simulink model "FAST_11To14_MPC"  (R2019a)
settings: Solver=FixedStepAuto  StartTime=0.0  StopTime=10*DT  FixedStep=DT  RelTol=1e-3
values from neighbouring files (symbols this model uses):
  Cq = 0.0 0.0 0.0 0.0 0.0 0.0 0.0 0.0 0.0 0.0 0.0 0.0 0.0 0.0 0.0 0.0 0.0 0.0 0.0 0.0 0.0 0.0 0.0 0.0 0.0 0.0 0.0 0.0 0.0 0.0 0.0 0.0 0.0 0.0 0.0 0.0 0.0 0.0 0.0 0.0 0.0 0.0 0.0 0.0 0.0 0.0 0.0 0.0 0.0 0.0 0.0 0.0 0.0 0.0 0.0 0.0 0.0 0.0 0.0 0.0 0.0 0.0 0.0 0.0 0.0 0.0 0.0 0.0 0.0 0.0 0.0 0.0 0.0 0.0 0.0 0.0 0.0 0.0 0.0 0.0 0.0 0.0 0.0 0.0 0.0 0.0 0.0 0.0 0.0 0.0 0.0 0.0 0.0 0.0 0.0 0.0 0.0 0.0 0.0 0.0    [DD_test.sldd]    (also in testOutList.m = saveVarsMat.Cq)
  Drivetrain = struct    [dataDLR.m]
  DT = 0.008    [dataDLR.m]    (also in generateReport.m; initLPVParam.m; initWorkspace.m; runCalculateEvalCriteria.m)
  Lin_points : value not decoded    [DD_test.sldd]
  mu_old = zeros(2*N*nu,1)    [testCtrl.m]
  Ng = 97    [dataDLR.m]    (also in testCtrl.m)
  omegabar = interp1(Lin_points.V,Lin_points.RSpeed,Vbar,'spline')    [testCtrl.m]
  OutList = OutTable.Properties.VariableNames    [initLPVParam.m]    (also in testCtrl.m; testOutList.m = cell(40, 1); testqLPV.m = cell(40, 1))
  U = zeros(2*N,1)    [testCtrl.m]
  xk = Xk(nxa+1:2*nxa)    [testCtrl.m]
  Xko = kron(ones(N,1),xk)    [testCtrl.m]
undefined symbols (not defined in the file or in its folder): Rotor_Lambda, Rotor_Lamda, Rotor_Pitch, strmatch
libraries: MdlLib_ProcessOutput x1
settings Model: ExtModeTrigMode=oneshot  ExtModeArmWhenConnect=off  Creator=Hazim Namik  LastModifiedBy=ditt_aj
settings DataIOCC: LimitDataPoints=on  SaveFormat=Array  ReturnWorkspaceOutputs=off
settings OptimizationCC: BlockReduction=off  BooleanDataType=off  LifeSpan=inf
settings DebuggingCC: SaveWithParameterizedLinksMsg=none  UnderspecifiedInitializationDetection=Classic  MergeDetectMultiDrivingBlocksExec=none  SignalResolutionControl=TryResolveAllWithWarning  SFUnexpectedBacktrackingDiag=warning  SFNoUnconditionalDefaultTransitionDiag=warning  SFExecutionAtInitializationDiag=none  ArithmeticOperatorsInVariantConditions=warning
settings HardwareCC: ProdBitPerPointer=32  ProdBitPerSizeT=32  ProdBitPerPtrDiffT=32  ProdLargestAtomicFloat=None  ProdIntDivRoundTo=Undefined  ProdEndianess=Unspecified  ProdWordSize=32  ProdHWDeviceType=32-bit Generic  TargetUnknown=on
settings ModelReferenceCC: PropagateSignalLabelsOutOfModel=off
settings SFSimCC: SimUseLocalCustomCode=off
settings RTWCC: RTWUseLocalCustomCode=off
settings CodeAppCC: StateflowObjectComments=on
settings GRTTargetCC: TargetLangStandard=C89/C90 (ANSI)  GeneratePreprocessorConditionals=Disable all
settings ConfigComp: CovMetricSettings=dw  CovHtmlReporting=on  CovSaveCumulativeToWorkspaceVar=on  CovSaveSingleToWorkspaceVar=on  CovExternalEMLEnable=off

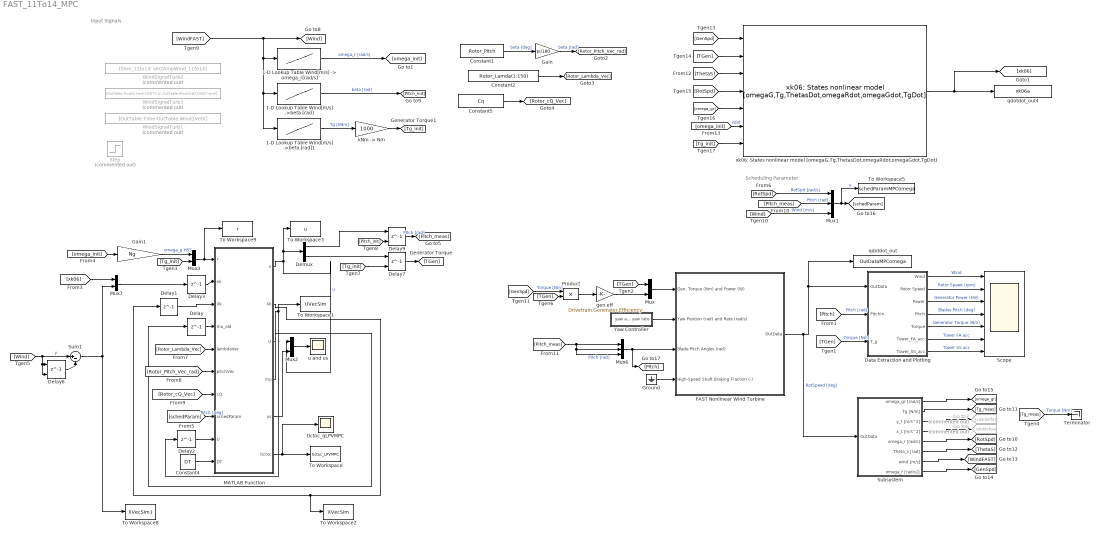
== system FAST_11To14_MPC ==
  note: Input Signals
  note: Scheduling Parameter
  "1-D Lookup Table Wind[m/s] -> omega_r[rad/s]" : Lookup_n-D  NumberOfTableDimensions=1  BreakpointsForDimension1=Lin_points.V  BreakpointsForDimension2=Rotor_Lambda  Table=Lin_points.RSpeed  InternalRulePriority=Speed  RndMeth=Simplest  InputSameDT=on
  1-D Lookup Table Wind[m/s] ->beta [rad] : Lookup_n-D  NumberOfTableDimensions=1  BreakpointsForDimension1=Lin_points.V  BreakpointsForDimension2=Rotor_Lambda  Table=Lin_points.Pitch  InternalRulePriority=Speed  RndMeth=Simplest  InputSameDT=on
  1-D Lookup Table Wind[m/s] ->beta [rad]1 : Lookup_n-D  NumberOfTableDimensions=1  BreakpointsForDimension1=Lin_points.V  BreakpointsForDimension2=Rotor_Lambda  Table=Lin_points.Torque  InternalRulePriority=Speed  RndMeth=Simplest  InputSameDT=on
  Constant1 : Constant  Value=Rotor_Pitch
  Constant2 : Constant  Value=Rotor_Lamda(1:150)
  Constant4 : Constant  Value=DT
  Constant5 : Constant  Value=Cq
  Data Extraction and Plotting : Subsystem
  Delay : Delay  DelayLength=1  InitialCondition=mu_old
  Delay1 : Delay  DelayLength=1  InitialCondition=Xko
  Delay2 : Delay  DelayLength=1  InitialCondition=U
  Delay3 : Delay  DelayLength=1  InitialCondition=xk
  Delay6 : Delay  DelayLength=1  InitialConditionSource=Input port  InitialCondition=[0, Lin_points.Torque(1)]
      settings: InputPortMap=u0,p4
  Delay7 : Delay  DelayLength=1  InitialConditionSource=Input port  InitialCondition=[0,omegabar]
      settings: InputPortMap=u0,p4
  Delay9 : Delay  DelayLength=1  InitialConditionSource=Input port  InitialCondition=[0,omegabar]
      settings: InputPortMap=u0,p4
  Demux : Demux  Outputs=2
  FAST Nonlinear Wind Turbine : Subsystem  mask(FAST Nonlinear Wind Turbine){}
      mask help: This block contains the FAST S-Function.
      mask init:
      | clear FAST_SFunc
  Gain : Gain  Gain=pi/180
  Gain1 : Gain  Gain=Ng
  Go to6 : Goto  Commented=on  GotoTag=xdotdotsw
  Go to7 : Goto  Commented=on  GotoTag=xdotdotfa
  Ground : Ground
  MATLAB Function : MATLAB Function  TreatAsAtomicUnit=on
  Mux{,2..3,7} (4 alike) : Mux  Inputs=2
  Mux1 : Mux  Inputs=3
  Mux6 : Mux  Inputs=3
  Product : Product  RndMeth=Zero
  Scope : Scope  NumInputPorts=7
      settings: Tag=Scope
  Step : Step  Commented=on  Time=0  Before=9.9960  After=11  SampleTime=0
  Subsystem : Subsystem
  Sum1 : Sum  Inputs=|+-
  Terminator : Terminator
  To Workspace : ToWorkspace  VariableName=tictoc_LPVMPC  SaveFormat=Timeseries  SampleTime=-1
  To Workspace1 : ToWorkspace  VariableName=UVecSim  SampleTime=-1
  To Workspace2 : ToWorkspace  VariableName=XVecSim  SampleTime=-1
  To Workspace3 : ToWorkspace  VariableName=u  SampleTime=-1
  To Workspace5 : ToWorkspace  VariableName=schedParamMPComega  SampleTime=-1
      settings: Save2DSignal=2-D array (concatenate along first dimension)
  To Workspace8 : ToWorkspace  VariableName=XVecSim1  SampleTime=-1
  To Workspace9 : ToWorkspace  VariableName=r  SampleTime=-1
  WindSignalTurb1 : FromWorkspace  Commented=on  VariableName=[OutTable.Time OutTable.Wind1VelX]  SampleTime=DT  OutputAfterFinalValue=Holding final value
  WindSignalTurb2 : FromWorkspace  Commented=on  VariableName=[time_11to14' vectAmpWind_11to14]  SampleTime=DT  OutputAfterFinalValue=Holding final value
  WindSignalTurb3 : FromWorkspace  Commented=on  VariableName=[OutTable.Time(1:(end-20/DT+1)),OutTable.Wind1VelX(20/DT:end)]  SampleTime=DT  OutputAfterFinalValue=Holding final value
  Yaw Controller : Subsystem
  gen eff : Gain  Gain=Drivetrain.Generator.Efficiency
  "kNm -> Nm" : Gain  Gain=1000
  qdotdot_out : ToWorkspace  VariableName=OutDataMPComega  SampleTime=-1
  qdotdot_out4 : ToWorkspace  VariableName=xk06a  SampleTime=-1
  tictoc_qLPVMPC : Scope
  u and us : Scope
  xk06: States nonlinear model [omegaG,Tg,ThetasDot,omegaRdot,omegaGdot,TgDot] : MdlLib_ProcessOutput/xk06: States nonlinear model [omegaG,Tg,ThetasDot,omegaRdot,omegaGdot,TgDot]  SystemSampleTime=-1
  wires:
  Mux/1 -> FAST Nonlinear Wind Turbine/1(Gen. Torque (Nm) and Power (W))
  Yaw Controller/1(yaw and yaw rate) -> FAST Nonlinear Wind Turbine/2(Yaw Position (rad) and Rate (rad/s))
  gen eff/1 -> Mux/2
  Product/1 -> gen eff/1
  Data Extraction and Plotting/3(Power) -> Scope/3  "Generator Power (kW)"
  [Pitch] -> Data Extraction and Plotting/2(PitchIn)  "Pitch [rad]"
  Data Extraction and Plotting/1(Wind) -> Scope/1  "Wind"
  Data Extraction and Plotting/2(Rotor Speed) -> Scope/2  "Rotor Speed (rpm)"
  [TGen] -> Data Extraction and Plotting/3(T_g)  "Torque [Nm]"
  Data Extraction and Plotting/4(Pitch) -> Scope/4  "Blades Pitch (deg)"
  Data Extraction and Plotting/5(Torque) -> Scope/5  "Generator Torque (Nm)"
  Data Extraction and Plotting/6(Tower_FA_acc) -> Scope/6  "Tower FA acc"
  Data Extraction and Plotting/7(Tower_SS_acc) -> Scope/7  "Tower SS acc"
  Ground/1 -> FAST Nonlinear Wind Turbine/4(High-Speed Shaft Braking Fraction (-))
  [TGen] -> Mux/1
  Delay3/1 -> MATLAB Function/2(xk)
  Mux7/1 -> Delay3/1
  MATLAB Function/3(U) -> Delay2/1, To Workspace1/1
  [omega_init] -> Gain1/1
  Sum1/1 -> To Workspace8/1, Mux7/2
  Gain1/1 -> Mux3/1  "omega_g HSS"
  Mux3/1 -> To Workspace9/1, MATLAB Function/1(r)
  [Wind] -> Delay6/2, Delay6/1, Sum1/1  "y"
  Delay6/1 -> Sum1/2
  [xk06] -> Mux7/1
  [Rotor_cQ_Vec] -> MATLAB Function/7(cQ)
  MATLAB Function/1(u) -> Demux/1, To Workspace3/1, Mux2/1  "u"
  Delay1/1 -> MATLAB Function/3("Xk ")
  [Tg_init] -> Mux3/2
  MATLAB Function/2(Xk) -> Delay1/1, To Workspace2/1
  [schedParam] -> MATLAB Function/8(schedParam)  "Pitch [deg]"
  Delay2/1 -> MATLAB Function/9("U ")
  Constant4/1 -> MATLAB Function/10(DT)
  MATLAB Function/6(tictoc) -> tictoc_qLPVMPC/1, To Workspace/1
  [Rotor_Lambda_Vec] -> MATLAB Function/5(lambdaVec)
  [Rotor_Pitch_Vec_rad] -> MATLAB Function/6(pitchVec)
  MATLAB Function/4(mu) -> Delay/1
  Delay/1 -> MATLAB Function/4(mu_old)
  MATLAB Function/5(us) -> Mux2/2
  Mux2/1 -> u and us/1
  Constant5/1 -> [Rotor_cQ_Vec]
  Gain/1 -> [Rotor_Pitch_Vec_rad]  "beta [rad]"
  "1-D Lookup Table Wind[m/s] -> omega_r[rad/s]"/1 -> [omega_init]  "omega_r [rad/s]"
  Constant1/1 -> Gain/1  "beta [deg]"
  1-D Lookup Table Wind[m/s] ->beta [rad]/1 -> [Pitch_init]  "beta [rad]"
  [WindFAST] -> [Wind], "1-D Lookup Table Wind[m/s] -> omega_r[rad/s]"/1, 1-D Lookup Table Wind[m/s] ->beta [rad]/1, 1-D Lookup Table Wind[m/s] ->beta [rad]1/1
  1-D Lookup Table Wind[m/s] ->beta [rad]1/1 -> "kNm -> Nm"/1  "Tg [kNm]"
  "kNm -> Nm"/1 -> [Tg_init]
  Constant2/1 -> [Rotor_Lambda_Vec]
  FAST Nonlinear Wind Turbine/1(OutData) -> Subsystem/1(OutData), qdotdot_out/1, Data Extraction and Plotting/1(OutData)  "RotSpeed [deg]"
  Delay7/1 -> [TGen]
  [Tg_init] -> Delay7/2
  [Pitch_meas] -> Mux6/1, Mux6/3, Mux6/2  "Pitch [rad]"
  Mux6/1 -> [Pitch], FAST Nonlinear Wind Turbine/3(Blade Pitch Angles (rad))
  [Pitch_init] -> Delay9/2
  Demux/2 -> Delay7/1
  Demux/1 -> Delay9/1
  [TGen] -> Product/2
  [GenSpd] -> Product/1  "Torque [Nm]"
  Delay9/1 -> [Pitch_meas]  "Pitch [rad]"
  [GenSpd] -> xk06: States nonlinear model [omegaG,Tg,ThetasDot,omegaRdot,omegaGdot,TgDot]/1
  [TGen] -> xk06: States nonlinear model [omegaG,Tg,ThetasDot,omegaRdot,omegaGdot,TgDot]/2
  [ThetaS] -> xk06: States nonlinear model [omegaG,Tg,ThetasDot,omegaRdot,omegaGdot,TgDot]/3
  [RotSpd] -> xk06: States nonlinear model [omegaG,Tg,ThetasDot,omegaRdot,omegaGdot,TgDot]/4
  [omega_gr] -> xk06: States nonlinear model [omegaG,Tg,ThetasDot,omegaRdot,omegaGdot,TgDot]/5
  [omega_init] -> xk06: States nonlinear model [omegaG,Tg,ThetasDot,omegaRdot,omegaGdot,TgDot]/6  "xdot"
  [Tg_init] -> xk06: States nonlinear model [omegaG,Tg,ThetasDot,omegaRdot,omegaGdot,TgDot]/7
  xk06: States nonlinear model [omegaG,Tg,ThetasDot,omegaRdot,omegaGdot,TgDot]/1 -> [xk06], qdotdot_out4/1
  Subsystem/2(Tg [N/m]) -> [Tg_meas]
  Subsystem/8(omega_r [rad/s]1) -> [GenSpd]
  Subsystem/7(wind [m/s]) -> [WindFAST]
  Subsystem/6(Theta_s [rad]) -> [ThetaS]
  Subsystem/1(omega_gr [rad/s]) -> [omega_gr]
  Subsystem/3(y_t [m/s^2]) -> Go to7/1
  Subsystem/5(omega_r [rad/s]) -> [RotSpd]
  Subsystem/4(x_t [m/s^2]) -> Go to6/1
  [Tg_meas] -> Terminator/1  "Torque [Nm]"
  [Pitch_meas] -> Mux1/2  "Pitch [rad]"
  Mux1/1 -> To Workspace5/1, [schedParam]  "y"
  [RotSpd] -> Mux1/1  "RotSpd [rad/s]"
  [Wind] -> Mux1/3  "Wind [m/s]"

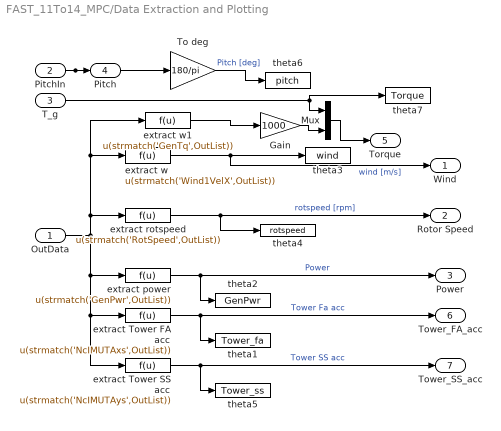
== system FAST_11To14_MPC/Data Extraction and Plotting ==
  OutData : Inport
  PitchIn : Inport  Port=2
  T_g : Inport  Port=3
  Gain : Gain  Gain=1000
  Mux : Mux  Inputs=2
  To deg : Gain  Gain=180/pi
  extract Tower FA acc : Fcn  Expr=u(strmatch('NcIMUTAxs',OutList))
  extract Tower SS acc : Fcn  Expr=u(strmatch('NcIMUTAys',OutList))
  extract power : Fcn  Expr=u(strmatch('GenPwr',OutList))
  extract rotspeed : Fcn  Expr=u(strmatch('RotSpeed',OutList))
  extract w : Fcn  Expr=u(strmatch('Wind1VelX',OutList))
  extract w1 : Fcn  Expr=u(strmatch('GenTq',OutList))
  theta1 : ToWorkspace  VariableName=Tower_fa  SampleTime=-1
      settings: MaxDataPoints=Inf  Decimation=3
  theta2 : ToWorkspace  VariableName=GenPwr  SampleTime=-1
      settings: MaxDataPoints=Inf  Decimation=3
  theta3 : ToWorkspace  VariableName=wind  SampleTime=-1
      settings: MaxDataPoints=Inf  Decimation=3
  theta4 : ToWorkspace  VariableName=rotspeed  SampleTime=-1
      settings: MaxDataPoints=Inf  Decimation=3
  theta5 : ToWorkspace  VariableName=Tower_ss  SampleTime=-1
      settings: MaxDataPoints=Inf  Decimation=3
  theta6 : ToWorkspace  VariableName=pitch  SampleTime=-1
      settings: MaxDataPoints=Inf  Decimation=3
  theta7 : ToWorkspace  VariableName=Torque  SampleTime=-1
      settings: MaxDataPoints=Inf  Decimation=3
  Wind : Outport
  Rotor Speed : Outport  Port=2
  Power : Outport  Port=3
  Pitch : Outport  Port=4
  Torque : Outport  Port=5
  Tower_FA_acc : Outport  Port=6
  Tower_SS_acc : Outport  Port=7
  wires:
  extract w/1 -> Wind/1, theta3/1  "wind [m/s]"
  extract rotspeed/1 -> theta4/1, Rotor Speed/1  "rotspeed [rpm]"
  extract power/1 -> theta2/1, Power/1  "Power"
  PitchIn/1 -> To deg/1, Pitch/1
  T_g/1 -> Mux/1, theta7/1
  extract Tower FA acc/1 -> theta1/1, Tower_FA_acc/1  "Tower Fa acc"
  OutData/1 -> extract w/1, extract w1/1, extract rotspeed/1, extract Tower SS acc/1, extract Tower FA acc/1, extract power/1
  extract Tower SS acc/1 -> theta5/1, Tower_SS_acc/1  "Tower SS acc"
  extract w1/1 -> Gain/1
  Gain/1 -> Mux/2
  Mux/1 -> Torque/1
  To deg/1 -> theta6/1  "Pitch [deg]"

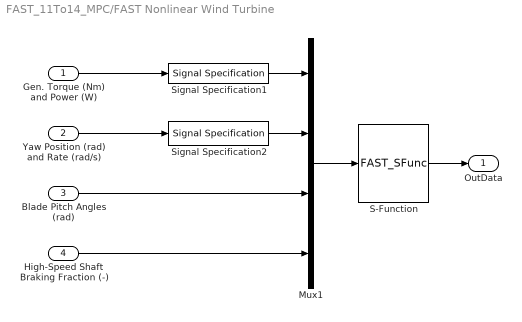
== system FAST_11To14_MPC/FAST Nonlinear Wind Turbine ==
  Gen. Torque (Nm) and Power (W) : Inport
  Yaw Position (rad) and Rate (rad/s) : Inport  Port=2
  Blade Pitch Angles (rad) : Inport  Port=3
  High-Speed Shaft Braking Fraction (-) : Inport  Port=4
  Mux1 : Mux
  S-Function : S-Function  FunctionName=FAST_SFunc  Parameters=FAST_InputFileName, TMax, 0  SFunctionDeploymentMode=off  EnableBusSupport=off
  Signal Specification1 : SignalSpecification  OutDataTypeStr=double  Dimensions=2
  Signal Specification2 : SignalSpecification  OutDataTypeStr=double  Dimensions=2
  OutData : Outport
  wires:
  Gen. Torque (Nm) and Power (W)/1 -> Signal Specification1/1
  S-Function/1 -> OutData/1
  Mux1/1 -> S-Function/1
  Blade Pitch Angles (rad)/1 -> Mux1/3
  Yaw Position (rad) and Rate (rad/s)/1 -> Signal Specification2/1
  Signal Specification1/1 -> Mux1/1
  Signal Specification2/1 -> Mux1/2
  High-Speed Shaft Braking Fraction (-)/1 -> Mux1/4

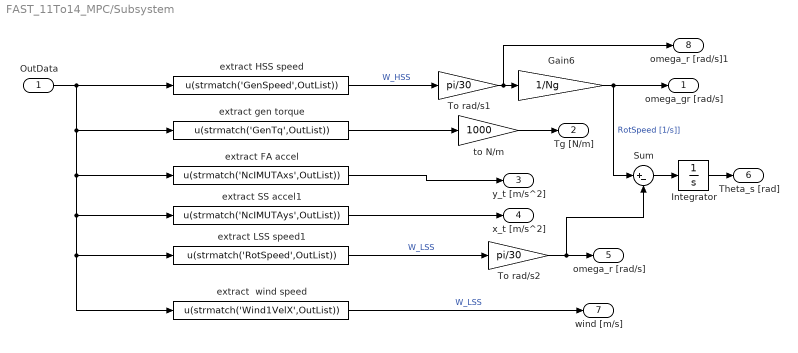
== system FAST_11To14_MPC/Subsystem ==
  OutData : Inport
  Gain6 : Gain  Gain=1/Ng
  Integrator : Integrator
  Sum : Sum  Inputs=|+-
  To rad/s1 : Gain  Gain=pi/30
  To rad/s2 : Gain  Gain=pi/30
  extract  wind speed : Fcn  Expr=u(strmatch('Wind1VelX',OutList))
  extract FA accel : Fcn  Expr=u(strmatch('NcIMUTAxs',OutList))
  extract HSS speed : Fcn  Expr=u(strmatch('GenSpeed',OutList))
  extract LSS speed1 : Fcn  Expr=u(strmatch('RotSpeed',OutList))
  extract SS accel1 : Fcn  Expr=u(strmatch('NcIMUTAys',OutList))
  extract gen torque : Fcn  Expr=u(strmatch('GenTq',OutList))
  to N/m : Gain  Gain=1000
  omega_gr [rad/s] : Outport
  Tg [N/m] : Outport  Port=2
  y_t [m/s^2] : Outport  Port=3
  x_t [m/s^2] : Outport  Port=4
  omega_r [rad/s] : Outport  Port=5
  Theta_s [rad] : Outport  Port=6
  wind [m/s] : Outport  Port=7
  omega_r [rad/s]1 : Outport  Port=8
  wires:
  to N/m/1 -> Tg [N/m]/1
  OutData/1 -> extract HSS speed/1, extract gen torque/1, extract  wind speed/1, extract LSS speed1/1, extract SS accel1/1, extract FA accel/1
  extract FA accel/1 -> y_t [m/s^2]/1
  extract HSS speed/1 -> To rad/s1/1  "W_HSS"
  extract gen torque/1 -> to N/m/1
  extract SS accel1/1 -> x_t [m/s^2]/1
  To rad/s1/1 -> omega_r [rad/s]1/1, Gain6/1
  extract LSS speed1/1 -> To rad/s2/1  "W_LSS"
  Gain6/1 -> omega_gr [rad/s]/1, Sum/1  "RotSpeed [1/s]]"
  To rad/s2/1 -> Sum/2, omega_r [rad/s]/1
  Sum/1 -> Integrator/1
  Integrator/1 -> Theta_s [rad]/1
  extract  wind speed/1 -> wind [m/s]/1  "W_LSS"

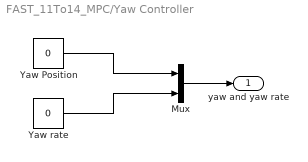
== system FAST_11To14_MPC/Yaw Controller ==
  Mux : Mux  Inputs=2
  Yaw Position : Constant  Value=0
  Yaw rate : Constant  Value=0
  yaw and yaw rate : Outport
  wires:
  Mux/1 -> yaw and yaw rate/1
  Yaw Position/1 -> Mux/1
  Yaw rate/1 -> Mux/2

== matlab function FAST_11To14_MPC/MATLAB Function ==
  settings: updateMethod=DISCRETE
  data: r input; u output; xk input; Xk input; mu_old input; lambdaVec input; pitchVec input; cQ input; schedParam input; U input; DT input; Xk output; U output; mu output; us output; tictoc output
function [u,Xk,U,mu,us,tictoc] = qLPVMPC_WECS(r,xk,Xk,mu_old,lambdaVec,pitchVec,cQ,schedParam,U,DT)
% MATLAB_Function calculates controller output u. It turns the QP into a 
% linear complementarity problem (LCP) and solves it with Lemke's algorithm.
%
% Inputs: * r: reference
%         * xk: quasiLPV KF state estimates
%         * Xk: Xko(= L*xk+S*U) delayed by one sample timestep
%         * mu_old: mu delayed by one sample timestep
%         * lambdaVec: lambda vector for cQ LUT 
%         * pitchVec: pitch vector for cQ LUT 
%         * cQ: torque coefficients LUT matrix
%         * schedParam: current values [omegaR, beta, V]
%         * U: U (from Xko = L*xk+S*U) delayed by one sample timestep
%
% Outputs: * u: controller output at current time step
%          * Xko: Future state trajectory (L*xk+S*U)
%          * U: Future input trajectory 
%          * mu: Result Lemke's algorithm/LCP: M mu +q >=0, mu>=0, mu'(Mmu+q)=0
%          * us: xuss(end) from xuss = [eye(4)-Ass -Bss;[1 0 0 0] 0]\[Bss*d;1]
%          * tictoc: tic-toc result

% Pablo S.G. Cisneros, Herbert Werner, ICS TUHH

%#codegen
coder.extrinsic('tic');
coder.extrinsic('toc');
tictoc = 0;
tic

%% Init N, Q, R
N = 40;
q_ = [1000 1 0 0*10^3 0*10^3 0 0]; %[10^4 0.1 1 1 100 0.1 0]; %q_ = [100 1000 1 0.01 0]; 7.351e+02 1.000e+00 1.938e+09 1.625e+08 1.491e+08 1.657e+03
r_ = [10^8 1]; %[10^7,0.1];
R_ = kron(eye(N),diag(r_)); %R_ = 1000*eye(N); 
p = 10*q_; %P = 1000*diag(q_);

Ulim = repmat([8 * pi/180, 20000]',2*N,1); %rate constraints 

Control_Pitch_Max = 90 /180 * pi;
Control_Pitch_Min = 0 /180 * pi;
Control_Torque_Limit = 47403;
Control_Torque_Min = 200;
schedParam(2) = min(max(schedParam(2), Control_Pitch_Min),Control_Pitch_Max);

% isBetaState = 0;
% nx = 4 + isBetaState; % number states plant: ThetaS,omegaR,omegaG,Tg
% ny = 2 + isBetaState; % number of outputs plant omegaG,Tg
nxA = 7;% nx + ny + 1; %number states augmented plant 
nu = 2; % plant inputs: Tg_ref, beta_ref

%% Shift Xk
Xk(1:end-nxA) = Xk(nxA+1:end); 
%Xk(1:nxA)

%% Calculate input u_dot_s = 0  and steady state x = r
us = [0;0]; %xuss(nxA+1:nxA+2); % xuss = [eye(size(Ass))-Ass -Bss;[1 0 0 0] 0] \ [Bss*d;reference];

iterations = 1; % omega_ref(Vest), Tg_ref(Vest)
refVec = zeros(nxA,1);
refVec(1:2) = r;
ref = repmat(refVec,N,1); %ref = kron(ones(N,1),[r; 0; 0; 0;0]);

for i = 1:iterations
    [L,S,H,g] = HSqLd_WT(N,q_,R_,p,xk,Xk,DT,ref,us,lambdaVec,pitchVec,cQ,schedParam,U);
    
    %% %%%%%%Turn QP into LCP and solve it%%%%%%%%%
    Ac_ = [-eye(N*nu);eye(N*nu)];
    bc_ = - Ulim;
    Hi = eye(size(H,1))/H;
    M = Ac_*Hi*Ac_';
    q = -Ac_*Hi*g - bc_;
 
    mu = lemke(M,q,mu_old);
 
    U = Hi*(Ac_'*mu-g);
    U(isnan(U)) = 0;
    
    %% %%%%%%%%%%%%%%%%%%%%%%%%%%%%%%%%%%%%%%%%%%%%    
    Xk = L*xk+S*U;
end

u =  [min( max(U(1) + schedParam(2), Control_Pitch_Min),Control_Pitch_Max),... % pitch
min(max(U(2) + Xk(2), Control_Torque_Min),Control_Torque_Limit)]'; % torque

tictoc = toc;

% For debugging
%%%%%%%%%%% Compute Hessian H, derivative g = dJk/dUk %%
% min Jk(Uk) s.t. h1(Uk) = 0, h2(Uk) < 0, at current estimate xl
% <=> min( x'H(xl)x + g(xl)x s.t. dh1(xl)x+h1(xl)=0, dh2(xl)x+h2(xl)< 0
% with 
% Jk = (Lx+SUk-Xss)'Q(Lx+SUk-Xss) +(Uk-Uss)'R(Uk-Uss) + Psi
% dJk/dUk = 2S'Q (Lx+SUk-Xss) + 2R(Uk-Uss) 

% diffX = Xk(1:(end - nxA)) - ref(1:(end -nxA));
% diffXEnd = Xk((end - nxA +1):end) - ref((end - nxA +1):end);
% 
% % Q_ = kron(eye(N-1),diag(q_));
% % Qcomp = diffX' * Q_ * diffX;
% % Pcomp = diffXEnd' * diag(p)* diffXEnd;
% % Rcomp = U' * R_ * U;
% 
% diffXMat = sum(reshape(diffX.^2, nxA, N-1),2);
% UMat = sum(reshape(U.^2, 2, N),2);
